simulink model "human_detection_navigation_system"  (R2025b)
settings: Solver=VariableStepAuto  StartTime=0.0  StopTime=10.0  RelTol=1e-3
libraries: simulink x1
settings Model: Creator=palellabhanuprasad  LastModifiedBy=palellabhanuprasad

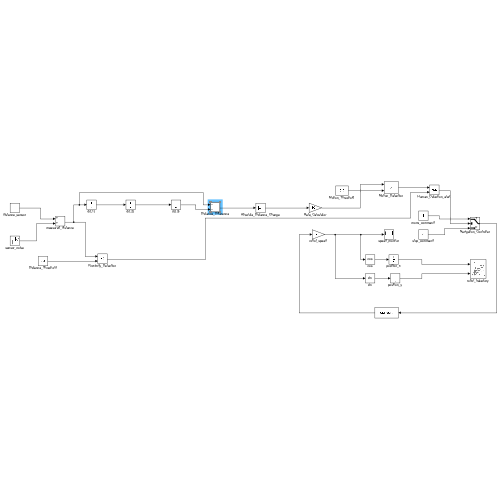
[thumbnail: Simulink's stored preview of the top-level diagram]
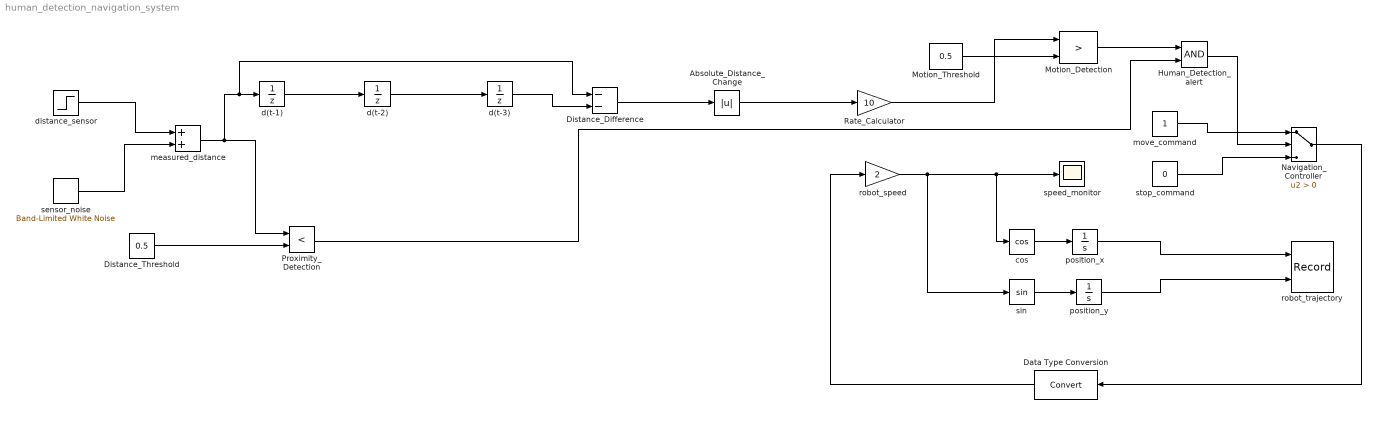
== system human_detection_navigation_system ==
  Absolute_Distance_Change : Abs  SaturateOnIntegerOverflow=off
  Data Type Conversion : DataTypeConversion  SaturateOnIntegerOverflow=off  RndMeth=Floor
  Distance_Difference : Sum  Inputs=--
  Distance_Threshold : Constant  Value=0.5
  Human_Detection_alert : Logic  AllPortsSameDT=off  OutDataTypeStr=boolean
  Motion_Detection : RelationalOperator  Operator=>  OutDataTypeStr=boolean  RndMeth=Simplest  InputSameDT=off
  Motion_Threshold : Constant  Value=0.5
  Navigation_Controller : Switch  Criteria=u2 > Threshold  SaturateOnIntegerOverflow=off  InputSameDT=off
  Proximity_Detection : RelationalOperator  Operator=<  OutDataTypeStr=boolean  RndMeth=Simplest  InputSameDT=off
  Rate_Calculator : Gain  Gain=10
  cos : Trigonometry  Operator=cos
  d(t-1) : UnitDelay  SampleTime=-1  HasFrameUpgradeWarning=on
  d(t-2) : UnitDelay  SampleTime=-1  HasFrameUpgradeWarning=on
  d(t-3) : UnitDelay  SampleTime=-1  HasFrameUpgradeWarning=on
  distance_sensor : Step  After=4  SampleTime=0
  measured_distance : Sum
  move_command : Constant
  position_x : Integrator
  position_y : Integrator
  robot_speed : Gain  Gain=2
  robot_trajectory : Record  NumPorts=2.0  FileSettingsInternal="{\"entries\":[{\"content\":{\"excelSettings\":{\"content\":{},\"type\":\"Streamout.ExcelSettings\"},\"parquetSettings\":{\"content\":{},\"type\":\"Streamout.ParquetSettings\"}},\"type\":\"Streamout.FileSettingStorage\",\"uuid\":\"\"}],\"packageUris\":[\"http:\\/\\/schema.mathworks.com\\/mf0\\/streamout_blocks\\/R2020a\"],\"version\":\"1.0\"}"  FrameSettings=[0, 0]  Layout=[1 1]  SignalsInternal="{\"entries\":[{\"content\":{\"signals\":[{\"content\":{\"blockPath\":[],\"dimensions\":[1],\"domain\":\"\",\"lineColor\":\"#a2142f\",\"plots\":[ 1 ],\"port\":1,\"sid\":[\"\"],\"signalID\":1,\"signalName\":\"position_x\"},\"type\":\"RecordBlkView.Signal\",\"uuid\":\"\"},{\"content\":{\"blockPath\":[],\"dimensions\":[1],\"domain\":\"\",\"lineColor\":\"#139fff\",\"plots\":[ 1 ],\"port\":2,\"sid\":[\"\"],\"signalID\":2,\"signalName\":\"position_y\"},\"type\":\"RecordBlkView.Signal\",\"uuid\":\"\"}]},\"type\":\"RecordBlkView.InputSignals\",\"uuid\":\"\"}],\"packageUris\":[\"http:\\/\\/schema.mathworks.com\\/mf0\\/streamout_blocks\\/R2020a\"],\"version\":\"1.0\"}"  VisualizationBindings="{\"xyplotplugin\":{\"info\":[{\"series\":[{\"bindingParametersList\":[{\"parameter\":\"X-Axis\",\"signalID\":1,\"signalName\":\"position_x\"},{\"parameter\":\"Y-Axis\",\"signalID\":2,\"signalName\":\"position_y\"}],\"seriesID\":0}],\"subplotID\":1}]}}"  CompatibilityTag=XY
  sensor_noise : simulink/Sources/Band-Limited White Noise  Cov=[0.1]  Ts=0.001  seed=[23341]
  sin : Trigonometry
  speed_monitor : Scope
      settings: ActiveDisplayYMinimum=-0.24999999999999994  ActiveDisplayYMaximum=2.25
  stop_command : Constant  Value=0
  wires:
  distance_sensor/1 -> measured_distance/1
  sensor_noise/1 -> measured_distance/2
  measured_distance/1 -> Proximity_Detection/1, Distance_Difference/1, d(t-1)/1
  d(t-1)/1 -> d(t-2)/1
  d(t-2)/1 -> d(t-3)/1
  d(t-3)/1 -> Distance_Difference/2
  Distance_Difference/1 -> Absolute_Distance_Change/1
  Absolute_Distance_Change/1 -> Rate_Calculator/1
  Rate_Calculator/1 -> Motion_Detection/1
  Motion_Threshold/1 -> Motion_Detection/2
  Distance_Threshold/1 -> Proximity_Detection/2
  Motion_Detection/1 -> Human_Detection_alert/1
  Proximity_Detection/1 -> Human_Detection_alert/2
  move_command/1 -> Navigation_Controller/1
  Human_Detection_alert/1 -> Navigation_Controller/2
  stop_command/1 -> Navigation_Controller/3
  robot_speed/1 -> sin/1, cos/1, speed_monitor/1
  cos/1 -> position_x/1
  sin/1 -> position_y/1
  position_x/1 -> robot_trajectory/1
  position_y/1 -> robot_trajectory/2
  Navigation_Controller/1 -> Data Type Conversion/1
  Data Type Conversion/1 -> robot_speed/1
